simulink model "model_new_visual"  (R2023a)
settings: Solver=VariableStepAuto  StartTime=0.0  StopTime=3  RelTol=1e-3
model workspace: external: MATLAB File model_new_DataFile.m (data not in the file)
values from neighbouring files (symbols this model uses):
  smiData = struct    [model_new_DataFile.m]
undefined symbols (not defined in the file or in its folder): _, ____, ____16, ____19, ____20, ____3, ____4, ____4X6X3, ____6, ____6X10X3, ____7X11X2, ______, ______1, ______2, ______3_________________________, _______1_________________________2_________________________________航发支架总装, ________, ________1, ________20__1____6, ________6, _________, __________, __________2, __________40160, __________6x16x5, ____________, ____________2, ____________3X1, ______________, ______________1X5, __________________, ___________________, ____________________20__26____4, ____________________25__25____5, __________________SULERCH, ______________A, __________A, __________B, ______A__6, _X2_4E1D6746_X0_, _X2_652F64915EA7_X0_, _X2_7535673A5B8988C5677F_X0_, _X2_8F74627F677F_X0_, _航发支架总装, _默认_sldprt, A25, a__________100, BZ, C, CONNECTOR_5MMCLOSED2PIN_MALE_1, D1, DIP_SWITCH_8PIN_VIC2_1, DYJN, EC, EE, FUS606_REF_1, GE4C, IPOS__________, LAF30, M3________ ... (+34)
libraries: sm_lib x987, nesl_utility x6, simulink x4
(part 1 of 18)
settings Model: Creator=Miao xinge  LastModifiedBy=simcoe

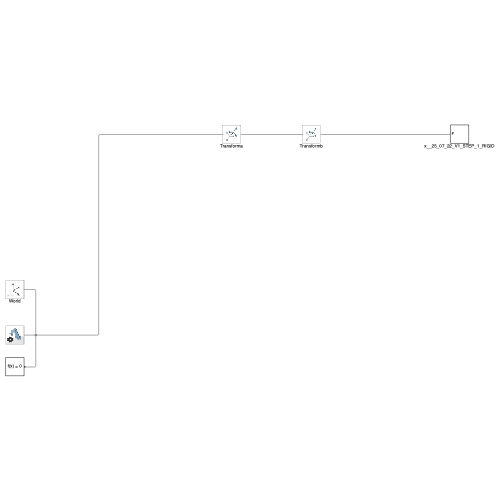
[thumbnail: Simulink's stored preview of the top-level diagram]
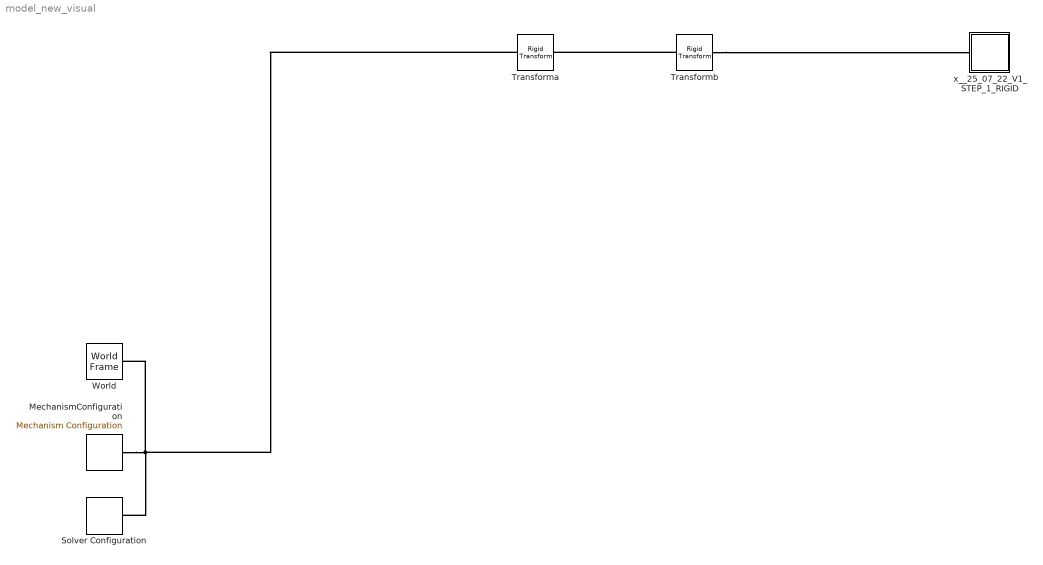
== system model_new_visual ==
  MechanismConfiguration : sm_lib/Utilities/Mechanism Configuration  UniformGravity=Constant  GravityVector=[0 -9.80665 0]  GravityVectorUnits=m/s^2  LinearizationDelta=0.001  JointModeTransitionNonlinearIterations=2
  Solver Configuration : nesl_utility/Solver Configuration  PhysicalDomain=network_engine_domain  SubClassName=solver  LeftPortType=input  RightPortType=generic  Tones=[]  Harmonics=[]  SimulateNoise=off  Profile=off  UseLocalSampling=off  EnableSwitchedLinearOptims=on  FrequencyDomain=off  UseCCode=off  RelTol=0.001  AbsTol=0.001  MinStep=1e-09  ToWorkspace=off  RevertToSquareIcSolve=off  NumHomotopyIterations=100  PhasorMode=off  PhasorModeNumHarmonics=1  ConsistencySolver=NEWTON_XTOL_AFTER_FTOL  IndexReductionMethod=DerivativeReplacement  DoDC=off  ResidualTolerance=1e-09  ConsistencyTolSource=GLOBAL  ConsistencyAbsTol=0.001  ConsistencyRelTol=0.001  ConsistencyTolFactor=0.001  UseLocalSolver=off  LocalSolverChoice=NE_BACKWARD_EULER_ADVANCER  ResolveIndetEquations=on  FunctionEvalNumThread=1  LocalSolverSampleTime=0.001  DoFixedCost=off  MaxNonlinIter=3  MaxModeIter=2  ComputeImpulses=off  ImpulseIterations=2  LinearAlgebra=auto  LinearAlgebraNumThread=0  EquationFormulation=NE_TIME_EF  DelaysMemoryBudget=1024  AutomaticFiltering=on  FilteringTimeConstant=0.001  PartitionStorageMethod=AS_NEEDED  PartitionMemoryBudget=1024  PartitionMethod=ROBUST
  Transforma : sm_lib/Frames and Transforms/Rigid Transform  TranslationMethod=Cartesian  TranslationStandardOffset=0  TranslationStandardOffsetUnits=m  TranslationStandardAxis=+Z  TranslationCartesianOffset=[ 0,0,0]  TranslationCartesianOffsetUnits=mm  TranslationROffset=0  TranslationROffsetUnits=m  TranslationZOffset=0  TranslationZOffsetUnits=m  TranslationThetaOffset=0  TranslationThetaOffsetUnits=deg  RotationMethod=ArbitraryAxis  RotationAngleUnits=rad  RotationStandardAxis=+Z  RotationAngle=0  RotationArbitraryAxis=[ 0,0,0]  FollAlignAxisA=+X  BaseAlignAxisA=+Y  FollAlignAxisB=+Y  BaseAlignAxisB=+Z  RotationSequenceAxes=FollowerAxes  RotationSequence=XYX  RotationSequenceAngles=[0 0 0]  RotationSequenceAnglesUnits=deg  RotationMatrix=[1 0 0; 0 1 0; 0 0 1]  Quaternion=[1 0 0 0]
  Transformb : sm_lib/Frames and Transforms/Rigid Transform  TranslationMethod=Cartesian  TranslationStandardOffset=0  TranslationStandardOffsetUnits=m  TranslationStandardAxis=+Z  TranslationCartesianOffset=smiData.RigidTransform(406).translation  TranslationCartesianOffsetUnits=mm  TranslationROffset=0  TranslationROffsetUnits=m  TranslationZOffset=0  TranslationZOffsetUnits=m  TranslationThetaOffset=0  TranslationThetaOffsetUnits=deg  RotationMethod=ArbitraryAxis  RotationAngleUnits=rad  RotationStandardAxis=+Z  RotationAngle=smiData.RigidTransform(406).angle  RotationArbitraryAxis=smiData.RigidTransform(406).axis  FollAlignAxisA=+X  BaseAlignAxisA=+Y  FollAlignAxisB=+Y  BaseAlignAxisB=+Z  RotationSequenceAxes=FollowerAxes  RotationSequence=XYX  RotationSequenceAngles=[0 0 0]  RotationSequenceAnglesUnits=deg  RotationMatrix=[1 0 0; 0 1 0; 0 0 1]  Quaternion=[1 0 0 0]
  World : sm_lib/Frames and Transforms/World Frame
  x__25_07_22_V1_STEP_1_RIGID : Subsystem
  connections:
  Transforma/LConn1 -- MechanismConfiguration/RConn1 -- Solver Configuration/RConn1 -- World/RConn1
  Transformb/RConn1 -- x__25_07_22_V1_STEP_1_RIGID/LConn1
  Transformb/LConn1 -- Transforma/RConn1
